simulink model "lab2"  (R2018a)
settings: Solver=ode45  StartTime=0.0  StopTime=10.0  MaxStep=0.001  RelTol=1e-10  AbsTol=1e-12
settings Model: Creator=Lora  LastModifiedBy=Lora

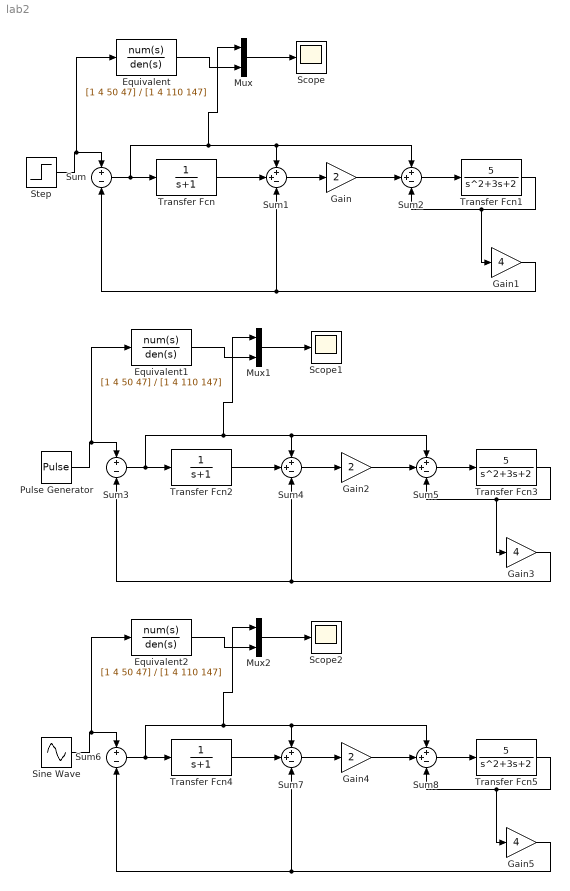
== system lab2 ==
  Equivalent : TransferFcn  Numerator=[1 4 50 47]  Denominator=[1 4 110 147]
  Equivalent1 : TransferFcn  Numerator=[1 4 50 47]  Denominator=[1 4 110 147]
  Equivalent2 : TransferFcn  Numerator=[1 4 50 47]  Denominator=[1 4 110 147]
  Gain : Gain  Gain=2
  Gain1 : Gain  Gain=4
  Gain2 : Gain  Gain=2
  Gain3 : Gain  Gain=4
  Gain4 : Gain  Gain=2
  Gain5 : Gain  Gain=4
  Mux : Mux  Inputs=2
  Mux1 : Mux  Inputs=2
  Mux2 : Mux  Inputs=2
  Pulse Generator : DiscretePulseGenerator  PulseType=Time based  Period=10  PulseWidth=5
  Scope : Scope
  Scope1 : Scope
  Scope2 : Scope
  Sine Wave : Sin  SampleTime=0
  Step : Step  SampleTime=0
  Sum : Sum  Inputs=+-
  Sum{1..2,4..5,7..8} (6 alike) : Sum  Inputs=++-
  Sum3 : Sum  Inputs=+-
  Sum6 : Sum  Inputs=+-
  Transfer Fcn : TransferFcn  Denominator=[1 1]
  Transfer Fcn1 : TransferFcn  Numerator=[5]  Denominator=[1 3 2]
  Transfer Fcn2 : TransferFcn  Denominator=[1 1]
  Transfer Fcn3 : TransferFcn  Numerator=[5]  Denominator=[1 3 2]
  Transfer Fcn4 : TransferFcn  Denominator=[1 1]
  Transfer Fcn5 : TransferFcn  Numerator=[5]  Denominator=[1 3 2]
  wires:
  Step/1 -> Equivalent/1, Sum/1
  Sum/1 -> Mux/1, Sum2/1, Sum1/1, Transfer Fcn/1
  Sum1/1 -> Gain/1
  Sum2/1 -> Transfer Fcn1/1
  Transfer Fcn/1 -> Sum1/2
  Gain/1 -> Sum2/2
  Transfer Fcn1/1 -> Gain1/1, Sum2/3
  Gain1/1 -> Sum1/3, Sum/2
  Equivalent/1 -> Mux/2
  Mux/1 -> Scope/1
  Transfer Fcn3/1 -> Gain3/1, Sum5/3
  Gain3/1 -> Sum4/3, Sum3/2
  Pulse Generator/1 -> Equivalent1/1, Sum3/1
  Mux1/1 -> Scope1/1
  Gain2/1 -> Sum5/2
  Equivalent1/1 -> Mux1/2
  Transfer Fcn2/1 -> Sum4/2
  Sum5/1 -> Transfer Fcn3/1
  Sum4/1 -> Gain2/1
  Sum3/1 -> Mux1/1, Sum5/1, Sum4/1, Transfer Fcn2/1
  Sum6/1 -> Mux2/1, Sum8/1, Sum7/1, Transfer Fcn4/1
  Sum7/1 -> Gain4/1
  Equivalent2/1 -> Mux2/2
  Sum8/1 -> Transfer Fcn5/1
  Gain4/1 -> Sum8/2
  Mux2/1 -> Scope2/1
  Gain5/1 -> Sum7/3, Sum6/2
  Sine Wave/1 -> Equivalent2/1, Sum6/1
  Transfer Fcn5/1 -> Gain5/1, Sum8/3
  Transfer Fcn4/1 -> Sum7/2
